simulink model "beaver_agent_env_ground_brake"  (R2022a)
settings: Solver=ode15s  StartTime=0.0  StopTime=30  FixedStep=1/120  MaxStep=0.005  RelTol=1e-6  AbsTol=1e-8
PreLoadFcn:
  | [aircraft, state] = astDehavillandBeaver();
  | thrustX = getCoefficient(aircraft,"CX","Propeller",Component="Propeller");
  | AileronCmd = 0.00202547955338193;
  | ElevatorCmd = -0.0109658218633661;
  | RudderCmd = -0.0374364069557001;
  | Throttle_Left = 0.16863024396043;
  | Throttle_Right = 0.16863024396043;
  | NoseWheelSteerCmdData = timeseries(0,0);
  | GearDownCmd = 1; RunwayMu = 0.65;
  | GroundMass = state.Mass;
  | GroundCrr = 0.015; GroundSideVGain = 0.35;
  | GroundYawGain = 0.15; GroundSteerGain = 0.8; NoseGearArm = 2.4;
  | 
  | Throttle_Left=0; Throttle_Right=0;
  | AileronCmd=0; ElevatorCmd=0; RudderCmd=0;
  | NoseWheelSteerCmdData=timeseries([0;0],[0;60]);
model workspace (MATLAB code in the model file + MAT data in the model file):
  GroundStatic.GearPositions = [2.4  0  1.5; -0.8  -1  1.5; -0.8  1  1.5]
  GroundStatic.RunwayZ = 0
  GroundStatic.StaticCompression = 0.06
  GroundStatic.InitialPosition = [0 0 -1.44]
  GroundStatic.InitialPositionOffset = [0 0 0]
  GroundStatic.InitialVelocity = [0 0 0]
  GroundStatic.InitialAttitude = [0 0 0]
  GroundStatic.InitialAngularRates = [0 0 0]
  GroundStatic.Mass = 2288.231
  GroundStatic.ReferenceGravity = 9.78032088963
  GroundStatic.LoadFractions = [0.25; 0.375; 0.375]
  GroundStatic.StaticWheelLoads = [5594.9083624; 8392.3625436; 8392.3625436]
  GroundStatic.NormalStiffness = [93248.4727066; 139872.70906; 139872.70906]
  GroundStatic.DampingRatio = 0.85
  GroundStatic.NormalDamping = [12416.2292263; 18624.3438394; 18624.3438394]
  GroundStatic.TireVelocityScale = 0.1
  GroundStatic.TireLateralCoefficient = 1
  GroundStatic.RollingCoefficient = 0.015
  GroundStatic.ParkingBrakeCoefficient = 0.5
  GroundStatic.ParkingBrakeCmd = 1
  GroundStatic.RunwayMu = 0.65
  GroundStatic.GearDown = 1
  GroundStatic.PowerOff = 1
  GroundStatic.AirSpeedFloor = 1
  GroundStatic.Description = 'Assumed three-point demonstration gear; replace with actual aircraft geometry/stiffness for performance use.'
  GroundStatic.LeftBrakeManual = 0
  GroundStatic.RightBrakeManual = 0
  GroundStatic.BrakeMode = 0
  GroundStatic.RunwayCenterlineYe = 0
  GroundStatic.RunwayCorrectionOnThreshold = 15.24
  GroundStatic.RunwayCorrectionOffThreshold = 3.048
  GroundStatic.RunwayCorrectionKp = 0.1
  GroundStatic.RunwayCorrectionKd = 0.5
  GroundStatic.DifferentialBrakeLimit = 1
  GroundStatic.BrakeCoefficient = 0.5
  GroundStatic.CorrectionRunwayAxis = 'Xe'
  GroundStatic.BrakeSystemMode = 1
  GroundStatic.AutoBrakePreArm = 0
  GroundStatic.AutoBrakeMinLevel = 0.15
  GroundStatic.NoseSteerLowSpeed = 2
  GroundStatic.NoseSteerHighSpeed = 20
  GroundStatic.NoseSteerAngleLowSpeed = 1.308996939
  GroundStatic.NoseSteerAngleHighSpeed = 0.10471975512
  inputs0.time = 0
  inputs0.signals(1).dimensions = 1
  inputs0.signals(1).values = -0.104711430294
  inputs0.signals(2).dimensions = 1
  inputs0.signals(2).values = -0.0698725229544
  inputs0.signals(3).dimensions = 1
  inputs0.signals(3).values = -0.000215042330254
  states.time = 0
  states.signals(1).values = 0
  states.signals(1).dimensions = 1
  states.signals(1).label = 'CSTATE'
  states.signals(1).blockName = 'untitled/6DOF EOM/6DOF (Euler Angles)/xe,ye,ze'
  states.signals(1).stateName = 'Xe'
  states.signals(1).inReferencedModel = 0
  states.signals(1).sampleTime = [0 0]
  states.signals(2).values = 0
  states.signals(2).dimensions = 1
  states.signals(2).label = 'CSTATE'
  states.signals(2).blockName = 'untitled/6DOF EOM/6DOF (Euler Angles)/xe,ye,ze'
  states.signals(2).stateName = 'Ye'
  states.signals(2).inReferencedModel = 0
  states.signals(2).sampleTime = [0 0]
  states.signals(3).values = -2202
  states.signals(3).dimensions = 1
  states.signals(3).label = 'CSTATE'
  states.signals(3).blockName = 'untitled/6DOF EOM/6DOF (Euler Angles)/xe,ye,ze'
  states.signals(3).stateName = 'Ze'
  states.signals(3).inReferencedModel = 0
  states.signals(3).sampleTime = [0 0]
  states.signals(4).values = 0.128665353089
  states.signals(4).dimensions = 1
  states.signals(4).label = 'CSTATE'
  states.signals(4).blockName = 'untitled/6DOF EOM/6DOF (Euler Angles)/Calculate DCM &
    | Euler Angles/phi
    | theta
    | psi'
  states.signals(4).stateName = 'phi'
  states.signals(4).inReferencedModel = 0
  states.signals(4).sampleTime = [0 0]
  states.signals(5).values = 0.259337659946
  states.signals(5).dimensions = 1
  states.signals(5).label = 'CSTATE'
  states.signals(5).blockName = 'untitled/6DOF EOM/6DOF (Euler Angles)/Calculate DCM &
    | Euler Angles/phi
    | theta
    | psi'
  states.signals(5).stateName = 'theta'
  states.signals(5).inReferencedModel = 0
  states.signals(5).sampleTime = [0 0]
  states.signals(6).values = -0.178947917154
  states.signals(6).dimensions = 1
  states.signals(6).label = 'CSTATE'
  states.signals(6).blockName = 'untitled/6DOF EOM/6DOF (Euler Angles)/Calculate DCM &
    | Euler Angles/phi
    | theta
    | psi'
  states.signals(6).stateName = 'psi'
  states.signals(6).inReferencedModel = 0
  states.signals(6).sampleTime = [0 0]
  states.signals(7).values = 36.9119692666
  states.signals(7).dimensions = 1
  states.signals(7).label = 'CSTATE'
  states.signals(7).blockName = 'untitled/6DOF EOM/6DOF (Euler Angles)/ub,vb,wb'
  states.signals(7).stateName = 'U'
  states.signals(7).inReferencedModel = 0
  states.signals(7).sampleTime = [0 0]
  states.signals(8).values = 8.10720863264
  states.signals(8).dimensions = 1
  states.signals(8).label = 'CSTATE'
  states.signals(8).blockName = 'untitled/6DOF EOM/6DOF (Euler Angles)/ub,vb,wb'
  states.signals(8).stateName = 'V'
  states.signals(8).inReferencedModel = 0
  states.signals(8).sampleTime = [0 0]
  states.signals(9).values = 8.82591882596
  states.signals(9).dimensions = 1
  states.signals(9).label = 'CSTATE'
  states.signals(9).blockName = 'untitled/6DOF EOM/6DOF (Euler Angles)/ub,vb,wb'
  states.signals(9).stateName = 'W'
  states.signals(9).inReferencedModel = 0
  states.signals(9).sampleTime = [0 0]
  states.signals(10).values = 0
  states.signals(10).dimensions = 1
  states.signals(10).label = 'CSTATE'
  states.signals(10).blockName = 'untitled/6DOF EOM/6DOF (Euler Angles)/p,q,r '
  states.signals(10).stateName = 'p'
  states.signals(10).inReferencedModel = 0
  states.signals(10).sampleTime = [0 0]
  states.signals(11).values = 0
  states.signals(11).dimensions = 1
  states.signals(11).label = 'CSTATE'
  states.signals(11).blockName = 'untitled/6DOF EOM/6DOF (Euler Angles)/p,q,r '
  states.signals(11).stateName = 'q'
  states.signals(11).inReferencedModel = 0
  states.signals(11).sampleTime = [0 0]
  states.signals(12).values = 0
  states.signals(12).dimensions = 1
  states.signals(12).label = 'CSTATE'
  states.signals(12).blockName = 'untitled/6DOF EOM/6DOF (Euler Angles)/p,q,r '
  states.signals(12).stateName = 'r'
  states.signals(12).inReferencedModel = 0
  states.signals(12).sampleTime = [0 0]
  states.signals(13).values = 0
  states.signals(13).dimensions = 1
  states.signals(13).label = 'CSTATE'
  states.signals(13).blockName = 'untitled/PID Controller/Integrator/Continuous/Integrator'
  states.signals(13).stateName = ''
  states.signals(13).inReferencedModel = 0
  states.signals(13).sampleTime = [0 0]
  states.signals(14).values = 0
  states.signals(14).dimensions = 1
  states.signals(14).label = 'CSTATE'
  states.signals(14).blockName = 'untitled/PID Controller/Filter/Cont. Filter/Filter'
  states.signals(14).stateName = ''
  states.signals(14).inReferencedModel = 0
  states.signals(14).sampleTime = [0 0]
  states.signals(15).values = 0
  states.signals(15).dimensions = 1
  states.signals(15).label = 'CSTATE'
  states.signals(15).blockName = 'untitled/PID Controller1/Integrator/Continuous/Integrator'
  states.signals(15).stateName = ''
  states.signals(15).inReferencedModel = 0
  states.signals(15).sampleTime = [0 0]
  states.signals(16).values = 0
  states.signals(16).dimensions = 1
  states.signals(16).label = 'CSTATE'
  states.signals(16).blockName = 'untitled/PID Controller1/Filter/Cont. Filter/Filter'
  states.signals(16).stateName = ''
  states.signals(16).inReferencedModel = 0
  states.signals(16).sampleTime = [0 0]
  states.signals(17).values = [0 0]
  states.signals(17).dimensions = 2
  states.signals(17).label = 'CSTATE'
  states.signals(17).blockName = 'untitled/Environment Model/Dryden Wind Turbulence Model 
    | (Continuous (+q +r))/Filters on velocities/Hwgw(s)/wg_p1'
  states.signals(17).stateName = ''
  states.signals(17).inReferencedModel = 0
  states.signals(17).sampleTime = [0 0]
  states.signals(18).values = [0 0]
  states.signals(18).dimensions = 2
  states.signals(18).label = 'CSTATE'
  states.signals(18).blockName = 'untitled/Environment Model/Dryden Wind Turbulence Model 
    | (Continuous (+q +r))/Filters on velocities/Hwgw(s)/wg_p2'
  states.signals(18).stateName = ''
  states.signals(18).inReferencedModel = 0
  states.signals(18).sampleTime = [0 0]
  states.signals(19).values = [0 0]
  states.signals(19).dimensions = 2
  states.signals(19).label = 'CSTATE'
  states.signals(19).blockName = 'untitled/Environment Model/Dryden Wind Turbulence Model 
    | (Continuous (+q +r))/Filters on velocities/Hvgw(s)/vg_p1'
  states.signals(19).stateName = ''
  states.signals(19).inReferencedModel = 0
  states.signals(19).sampleTime = [0 0]
  states.signals(20).values = [0 0]
  states.signals(20).dimensions = 2
  states.signals(20).label = 'CSTATE'
  states.signals(20).blockName = 'untitled/Environment Model/Dryden Wind Turbulence Model 
    | (Continuous (+q +r))/Filters on velocities/Hvgw(s)/vgw_p2'
  states.signals(20).stateName = ''
  states.signals(20).inReferencedModel = 0
  states.signals(20).sampleTime = [0 0]
  states.signals(21).values = [0 0]
  states.signals(21).dimensions = 2
  states.signals(21).label = 'CSTATE'
  states.signals(21).blockName = 'untitled/Environment Model/Dryden Wind Turbulence Model 
    | (Continuous (+q +r))/Filters on velocities/Hugw(s)/ug_p'
  states.signals(21).stateName = ''
  states.signals(21).inReferencedModel = 0
  states.signals(21).sampleTime = [0 0]
  states.signals(22).values = [0 0]
  states.signals(22).dimensions = 2
  states.signals(22).label = 'CSTATE'
  states.signals(22).blockName = 'untitled/Environment Model/Dryden Wind Turbulence Model 
    | (Continuous (+q +r))/Filters on angular rates/Hrgw/rgw_p'
  states.signals(22).stateName = ''
  states.signals(22).inReferencedModel = 0
  states.signals(22).sampleTime = [0 0]
  states.signals(23).values = [0 0]
  states.signals(23).dimensions = 2
  states.signals(23).label = 'CSTATE'
  states.signals(23).blockName = 'untitled/Environment Model/Dryden Wind Turbulence Model 
    | (Continuous (+q +r))/Filters on angular rates/Hqgw/qgw_p'
  states.signals(23).stateName = ''
  states.signals(23).inReferencedModel = 0
  states.signals(23).sampleTime = [0 0]
  states.signals(24).values = [0 0]
  states.signals(24).dimensions = 2
  states.signals(24).label = 'CSTATE'
  states.signals(24).blockName = 'untitled/Environment Model/Dryden Wind Turbulence Model 
    | (Continuous (+q +r))/Filters on angular rates/Hpgw/pgw_p'
  states.signals(24).stateName = ''
  states.signals(24).inReferencedModel = 0
  states.signals(24).sampleTime = [0 0]
  states0.time = 0
  states0.signals(1).values = [0 0 -2202]
  states0.signals(1).dimensions = 3
  states0.signals(1).label = 'CSTATE'
  states0.signals(1).blockName = 'asb6DOFAirframeTemplate/6DOF EOM/6DOF (Euler Angles)/xe,ye,ze'
  states0.signals(1).stateName = ''
  states0.signals(1).inReferencedModel = 0
  states0.signals(1).sampleTime = [0 0]
  states0.signals(2).values = [0.128665353089 0.259337659946 -0.178947917154]
  states0.signals(2).dimensions = 3
  states0.signals(2).label = 'CSTATE'
  states0.signals(2).blockName = 'asb6DOFAirframeTemplate/6DOF EOM/6DOF (Euler Angles)/Calculate DCM &
    | Euler Angles/phi
    | theta
    | psi'
  states0.signals(2).stateName = ''
  states0.signals(2).inReferencedModel = 0
  states0.signals(2).sampleTime = [0 0]
  states0.signals(3).values = [36.9119692666 8.10720863264 8.82591882596]
  states0.signals(3).dimensions = 3
  states0.signals(3).label = 'CSTATE'
  states0.signals(3).blockName = 'asb6DOFAirframeTemplate/6DOF EOM/6DOF (Euler Angles)/ub,vb,wb'
  states0.signals(3).stateName = ''
  states0.signals(3).inReferencedModel = 0
  states0.signals(3).sampleTime = [0 0]
  states0.signals(4).values = [0 0 0]
  states0.signals(4).dimensions = 3
  states0.signals(4).label = 'CSTATE'
  states0.signals(4).blockName = 'asb6DOFAirframeTemplate/6DOF EOM/6DOF (Euler Angles)/p,q,r '
  states0.signals(4).stateName = ''
  states0.signals(4).inReferencedModel = 0
  states0.signals(4).sampleTime = [0 0]
  states0.signals(5).values = [0 0]
  states0.signals(5).dimensions = 2
  states0.signals(5).label = 'CSTATE'
  states0.signals(5).blockName = 'asb6DOFAirframeTemplate/Environment Model/Dryden Wind Turbulence Model 
    | (Continuous (+q +r))/Filters on velocities/Hwgw(s)/wg_p1'
  states0.signals(5).stateName = ''
  states0.signals(5).inReferencedModel = 0
  states0.signals(5).sampleTime = [0 0]
  states0.signals(6).values = [0 0]
  states0.signals(6).dimensions = 2
  states0.signals(6).label = 'CSTATE'
  states0.signals(6).blockName = 'asb6DOFAirframeTemplate/Environment Model/Dryden Wind Turbulence Model 
    | (Continuous (+q +r))/Filters on velocities/Hwgw(s)/wg_p2'
  states0.signals(6).stateName = ''
  states0.signals(6).inReferencedModel = 0
  states0.signals(6).sampleTime = [0 0]
  states0.signals(7).values = [0 0]
  states0.signals(7).dimensions = 2
  states0.signals(7).label = 'CSTATE'
  states0.signals(7).blockName = 'asb6DOFAirframeTemplate/Environment Model/Dryden Wind Turbulence Model 
    | (Continuous (+q +r))/Filters on velocities/Hvgw(s)/vg_p1'
  states0.signals(7).stateName = ''
  states0.signals(7).inReferencedModel = 0
  states0.signals(7).sampleTime = [0 0]
  states0.signals(8).values = [0 0]
  states0.signals(8).dimensions = 2
  states0.signals(8).label = 'CSTATE'
  states0.signals(8).blockName = 'asb6DOFAirframeTemplate/Environment Model/Dryden Wind Turbulence Model 
    | (Continuous (+q +r))/Filters on velocities/Hvgw(s)/vgw_p2'
  states0.signals(8).stateName = ''
  states0.signals(8).inReferencedModel = 0
  states0.signals(8).sampleTime = [0 0]
  states0.signals(9).values = [0 0]
  states0.signals(9).dimensions = 2
  states0.signals(9).label = 'CSTATE'
  states0.signals(9).blockName = 'asb6DOFAirframeTemplate/Environment Model/Dryden Wind Turbulence Model 
    | (Continuous (+q +r))/Filters on velocities/Hugw(s)/ug_p'
  states0.signals(9).stateName = ''
  states0.signals(9).inReferencedModel = 0
  states0.signals(9).sampleTime = [0 0]
  states0.signals(10).values = [0 0]
  states0.signals(10).dimensions = 2
  states0.signals(10).label = 'CSTATE'
  states0.signals(10).blockName = 'asb6DOFAirframeTemplate/Environment Model/Dryden Wind Turbulence Model 
    | (Continuous (+q +r))/Filters on angular rates/Hrgw/rgw_p'
  states0.signals(10).stateName = ''
  states0.signals(10).inReferencedModel = 0
  states0.signals(10).sampleTime = [0 0]
  states0.signals(11).values = [0 0]
  states0.signals(11).dimensions = 2
  states0.signals(11).label = 'CSTATE'
  states0.signals(11).blockName = 'asb6DOFAirframeTemplate/Environment Model/Dryden Wind Turbulence Model 
    | (Continuous (+q +r))/Filters on angular rates/Hqgw/qgw_p'
  states0.signals(11).stateName = ''
  states0.signals(11).inReferencedModel = 0
  states0.signals(11).sampleTime = [0 0]
  states0.signals(12).values = [0 0]
  states0.signals(12).dimensions = 2
  states0.signals(12).label = 'CSTATE'
  states0.signals(12).blockName = 'asb6DOFAirframeTemplate/Environment Model/Dryden Wind Turbulence Model 
    | (Continuous (+q +r))/Filters on angular rates/Hpgw/pgw_p'
  states0.signals(12).stateName = ''
  states0.signals(12).inReferencedModel = 0
  states0.signals(12).sampleTime = [0 0]
  other statements: initialize6DOFSkyHogg;
values from neighbouring files (symbols this model uses):
  r = vec(out.r)    [ground_realtime_worker.m]    (also in probe_brake_correction.m; verify_ground_brake_model.m = runCase('turn_right_10',g,10,8))
  state = squeeze(controls.Data)    [finalize_ground_capability_checks.m]    (also in run_ground_capability_checks.m)
undefined symbols (not defined in the file or in its folder): aircraft, Earth, F, Light, MIL, WGS84
libraries: simulink x5, shared6dof x1, aerolibadyn x1, aerolibasang x1, aerolibatmos2 x1, aerolibwind2 x1, aerolibtransform2 x1, sharedtransform x1
(part 1 of 3)
settings Model: Creator=Petrichor  LastModifiedBy=velpro
settings SolverCC: AlgebraicLoopSolver=TrustRegion  AutoInsertRateTranBlk=on  InsertRTBMode=Never (minimum delay)  MinimalZcImpactIntegration=on  MaxZcPerStep=1
settings DataIOCC: ExternalInput=inputs0  InitialState=states  SaveFinalState=on  SaveFormat=Array  SaveState=on  LoggingToFile=on
settings OptimizationCC: EnhancedBackFolding=on  StrengthReduction=on  InitFltsAndDblsToZero=on  DifferentSizesBufferReuse=on
settings DebuggingCC: WriteAfterWriteMsg=DisableAll  AlgebraicLoopMsg=none  FcnCallInpInsideContextMsg=warning  UniqueDataStoreMsg=error  RootOutportRequireBusObject=none  StateNameClashWarn=warning  StrictBusMsg=ErrorOnBusTreatedAsVector  SFUnexpectedBacktrackingDiag=warning  SFNoUnconditionalDefaultTransitionDiag=warning  SFExecutionAtInitializationDiag=none  SFMachineParentedDataDiag=warning  ArithmeticOperatorsInVariantConditions=warning
settings ModelReferenceCC: PropagateSignalLabelsOutOfModel=off
settings SFSimCC: SimUseLocalCustomCode=off
settings RTWCC: RTWUseLocalCustomCode=off  DLArmComputeVersion=19.05
settings CodeAppCC: StateflowObjectComments=on

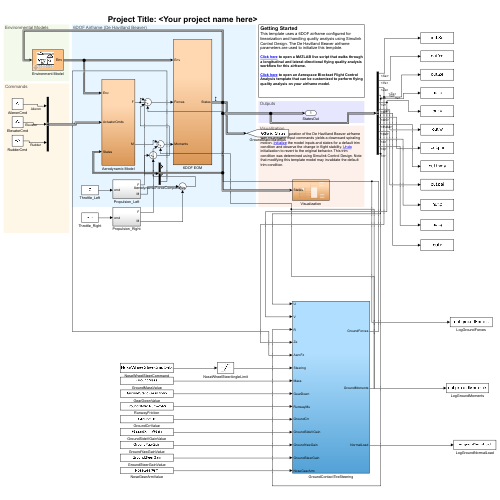
[thumbnail: Simulink's stored preview of the top-level diagram]
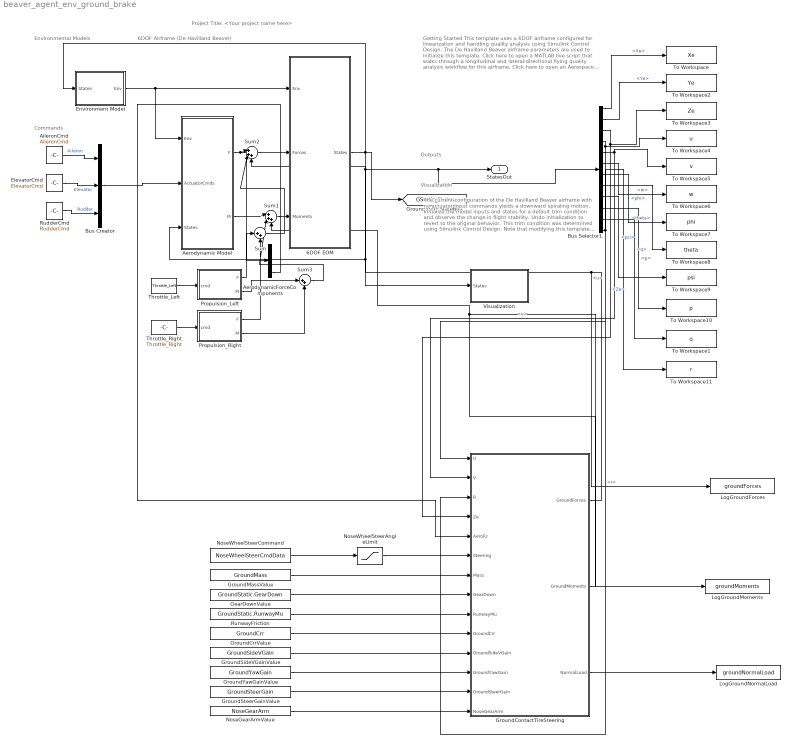
== system beaver_agent_env_ground_brake ==
  note: Project Title: <Your project name here>
  note: 6DOF Airframe (De Havilland Beaver)
  note: Environmental Models
  note: Commands
  note: The current configuration of the De Havilland Beaver airframe with no actuator input commands yields a downward spiraling motion. Initialize the model inputs and states for a default trim condition and observe the change in flight stability. Undo initialization to revert to the original behavior. This trim condition was determined using Simulink Control Design. Note that modifying this template model may invalidate the default trim condition.
  note: Visualization
  note: Outputs
  note: Getting Started
      | This template uses a 6DOF airframe configured for linearization and handling quality analysis using Simulink Control Design. The De Havilland Beaver airframe parameters are used to initialize this template.
      |
      | Click here to open a MATLAB live script that walks through a longitudinal and lateral-directional flying quality analysis workflow for this airframe.
      |
      | Click here to open an Aerospace Blockset Flight Control Analysis template that can be customized to perform flying quality analysis on your airframe model.
  6DOF EOM : Subsystem  VariantControl=eom3DOF
  Aerodynamic Model : Subsystem  VariantControl=aeroCONST
  AerodynamicForceComponents : Demux  Outputs=3
  AileronCmd : Constant  Value=AileronCmd
  Bus Creator : BusCreator  Inputs=3
  Bus Selector1 : BusSelector  OutputSignals=Xe,Ye,Ze,u,v,w,phi,theta,psi,p,q,r
  ElevatorCmd : Constant  Value=ElevatorCmd
  Environment Model : Subsystem  mask(Environment Model){spec=MIL-F-8785C, model=Continuous Dryden (+q -r), W20=5, Wdeg=0, TurbProb=10^-2 - Light, L_high=533.4, Wingspan=4, ts=0.1, Seed=[23341 23342 23343 23344], T_on=off, refAlt=state.GroundHeight}
      mask prompts: spec "aeroblks:aeroblkwind:blockWindTurbulenceModelParamSpecification"; model "aeroblks:aeroblkwind:blockWindTurbulenceModelParamModeltype"; W20 "Wind speed at 6 m defines the low-altitude intensity (m/s):"; Wdeg "Wind direction at 6 m (degrees clockwise from north):"; TurbProb "aeroblks:aeroblkwind:blockWindTurbulenceModelParamProbabilityofexceedanceofhighaltitudeintensity"; L_high "Scale length at medium/high altitudes (m):"; Wingspan "Wingspan (m):"; ts "Band limited noise sample time (sec):"; Seed "aeroblks:aeroblkwind:blockWindTurbulenceModelParamNoiseseedsugvgwgpg"; T_on "aeroblks:aeroblkwind:blockWindTurbulenceModelParamTurbulenceon"; refAlt "Reference height from Earth's surface to Flat Earth frame [m]:"
      mask help: This block contains an athmospheric model, a wind turbulence model, and a gravity model.
      mask Help: helpview(fullfile(docroot,'toolbox','aeroblks','aeroblks.map'), 'environment1');
      mask TypeOptions spec:
      | Dryden Wind Turbulence Model
      | (Continuous (+q +r))/spec
      mask TypeOptions model:
      | Dryden Wind Turbulence Model
      | (Continuous (+q +r))/model
      mask TypeOptions W20:
      | Dryden Wind Turbulence Model
      | (Continuous (+q +r))/W20
      mask TypeOptions Wdeg:
      | Dryden Wind Turbulence Model
      | (Continuous (+q +r))/Wdeg
      mask TypeOptions TurbProb:
      | Dryden Wind Turbulence Model
      | (Continuous (+q +r))/TurbProb
      mask TypeOptions L_high:
      | Dryden Wind Turbulence Model
      | (Continuous (+q +r))/L_high
      mask TypeOptions Wingspan:
      | Dryden Wind Turbulence Model
      | (Continuous (+q +r))/Wingspan
      mask TypeOptions ts:
      | Dryden Wind Turbulence Model
      | (Continuous (+q +r))/ts
      mask TypeOptions Seed:
      | Dryden Wind Turbulence Model
      | (Continuous (+q +r))/Seed
      mask TypeOptions T_on:
      | Dryden Wind Turbulence Model
      | (Continuous (+q +r))/T_on
      mask DialogControl Container4 Prompt: Atmospheric Model
      mask DialogControl Container17 Prompt: 1976 COESA-extended U.S. Standard Atmospheric Model
      mask DialogControl Control6 Prompt: There are no modifiable parameters for COESA.
      mask DialogControl Container6 Prompt: Wind Model
      mask DialogControl Container16 Prompt: Dryden Wind Turbulence Model
      mask DialogControl spec Prompt: Specification:
      mask DialogControl model Prompt: Model type:
      mask DialogControl TurbProb Prompt: Probability of exceedance of high-altitude intensity:
      mask DialogControl Seed Prompt: Noise seeds [ug vg wg pg]:
      mask DialogControl T_on Prompt: Turbulence on
      mask DialogControl Container8 Prompt: Gravity Model
      mask DialogControl Container18 Prompt: World Geodetic System (WGS 84) Gravity Taylor Series Model
      mask Display:
      | image('aeroenvironment.bmp',[.15,.15,.55,.75])
      | port_label('output',1,'Env')
  GearDownValue : Constant  Value=GroundStatic.GearDown
  GroundContactTireSteering : Subsystem
  GroundCrrValue : Constant  Value=GroundCrr
  GroundMassValue : Constant  Value=GroundMass
  GroundSideVGainValue : Constant  Value=GroundSideVGain
  GroundSteerGainValue : Constant  Value=GroundSteerGain
  GroundYawGainValue : Constant  Value=GroundYawGain
  LogGroundForces : ToWorkspace  VariableName=groundForces  SaveFormat=Timeseries  SampleTime=-1
  LogGroundMoments : ToWorkspace  VariableName=groundMoments  SaveFormat=Timeseries  SampleTime=-1
  LogGroundNormalLoad : ToWorkspace  VariableName=groundNormalLoad  SaveFormat=Timeseries  SampleTime=-1
  NoseGearArmValue : Constant  Value=NoseGearArm
  NoseWheelSteerAngleLimit : Saturate  UpperLimit=1.308996939  LowerLimit=-1.308996939
  NoseWheelSteerCommand : FromWorkspace  VariableName=NoseWheelSteerCmdData  Interpolate=off  OutputAfterFinalValue=Holding final value
  Propulsion_Left : Subsystem
      settings: RTWSystemCode=Inline
  Propulsion_Right : Subsystem
      settings: RTWSystemCode=Inline
  RudderCmd : Constant  Value=RudderCmd
  RunwayFriction : Constant  Value=GroundStatic.RunwayMu
  Sum : Sum  Inputs=|++
  Sum1 : Sum  Inputs=|+++  InputSameDT=on  SaturateOnIntegerOverflow=on  OutDataTypeStr=Inherit: Same as first input
  Sum2 : Sum  Inputs=|+++  InputSameDT=on  SaturateOnIntegerOverflow=on  OutDataTypeStr=Inherit: Same as first input
  Sum3 : Sum  Inputs=|++
  Throttle_Left : Constant  Value=Throttle_Left
  Throttle_Right : Constant  Value=Throttle_Right
  To Workspace : ToWorkspace  VariableName=Xe  SaveFormat=Timeseries  SampleTime=-1
  To Workspace1 : ToWorkspace  VariableName=q  SaveFormat=Timeseries  SampleTime=-1
  To Workspace10 : ToWorkspace  VariableName=p  SaveFormat=Timeseries  SampleTime=-1
  To Workspace11 : ToWorkspace  VariableName=r  SaveFormat=Timeseries  SampleTime=-1
  To Workspace2 : ToWorkspace  VariableName=Ye  SaveFormat=Timeseries  SampleTime=-1
  To Workspace3 : ToWorkspace  VariableName=Ze  SaveFormat=Timeseries  SampleTime=-1
  To Workspace4 : ToWorkspace  VariableName=u  SaveFormat=Timeseries  SampleTime=-1
  To Workspace5 : ToWorkspace  VariableName=v  SaveFormat=Timeseries  SampleTime=-1
  To Workspace6 : ToWorkspace  VariableName=w  SaveFormat=Timeseries  SampleTime=-1
  To Workspace7 : ToWorkspace  VariableName=phi  SaveFormat=Timeseries  SampleTime=-1
  To Workspace8 : ToWorkspace  VariableName=theta  SaveFormat=Timeseries  SampleTime=-1
  To Workspace9 : ToWorkspace  VariableName=psi  SaveFormat=Timeseries  SampleTime=-1
  Visualization : Subsystem
  StatesOut : Outport  OutDataTypeStr=double  VectorParamsAs1DForOutWhenUnconnected=off
  tag scope: GStatic_States=global
  wires:
  AileronCmd/1 -> Bus Creator/1  "Aileron"
  RudderCmd/1 -> Bus Creator/3  "Rudder"
  Sum2/1 -> 6DOF EOM/2(Forces)
  Sum1/1 -> 6DOF EOM/3(Moments)
  Aerodynamic Model/1(F) -> Sum2/1, AerodynamicForceComponents/1
  Aerodynamic Model/2(M) -> Sum1/1
  Environment Model/1(Env) -> 6DOF EOM/1(Env), Aerodynamic Model/1(Env)
  Bus Creator/1 -> Aerodynamic Model/2(ActuatorCmds)
  Propulsion_Left/1(F) -> Sum/1
  Propulsion_Right/1(F) -> Sum/2
  Sum/1 -> Sum2/2
  Propulsion_Left/2(M) -> Sum3/1
  Propulsion_Right/2(M) -> Sum3/2
  Sum3/1 -> Sum1/2
  ElevatorCmd/1 -> Bus Creator/2  "Elevator"
  Throttle_Left/1 -> Propulsion_Left/1(cmd)
  Throttle_Right/1 -> Propulsion_Right/1(cmd)
  Bus Selector1/4 -> To Workspace4/1, GroundContactTireSteering/1(U)  "<u>"
  Bus Selector1/6 -> To Workspace6/1  "<w>"
  Bus Selector1/10 -> To Workspace10/1  "<p>"
  Bus Selector1/11 -> To Workspace1/1  "<q>"
  Bus Selector1/7 -> To Workspace7/1  "<phi>"
  Bus Selector1/1 -> To Workspace/1  "<Xe>"
  Bus Selector1/9 -> To Workspace9/1  "<psi>"
  Bus Selector1/2 -> To Workspace2/1  "<Ye>"
  6DOF EOM/1(States) -> [GStatic_States], Environment Model/1(States), Bus Selector1/1, StatesOut/1, Aerodynamic Model/3(States), Visualization/1(States)
  Bus Selector1/8 -> To Workspace8/1  "<theta>"
  Bus Selector1/12 -> To Workspace11/1, GroundContactTireSteering/3(R)  "<r>"
  Bus Selector1/5 -> To Workspace5/1, GroundContactTireSteering/2(V)  "<v>"
  Bus Selector1/3 -> To Workspace3/1, GroundContactTireSteering/4(Ze)  "<Ze>"
  NoseWheelSteerCommand/1 -> NoseWheelSteerAngleLimit/1
  AerodynamicForceComponents/3 -> GroundContactTireSteering/5(AeroFz)
  NoseWheelSteerAngleLimit/1 -> GroundContactTireSteering/6(Steering)
  GroundMassValue/1 -> GroundContactTireSteering/7(Mass)
  GearDownValue/1 -> GroundContactTireSteering/8(GearDown)
  RunwayFriction/1 -> GroundContactTireSteering/9(RunwayMu)
  GroundCrrValue/1 -> GroundContactTireSteering/10(GroundCrr)
  GroundSideVGainValue/1 -> GroundContactTireSteering/11(GroundSideVGain)
  GroundYawGainValue/1 -> GroundContactTireSteering/12(GroundYawGain)
  GroundSteerGainValue/1 -> GroundContactTireSteering/13(GroundSteerGain)
  NoseGearArmValue/1 -> GroundContactTireSteering/14(NoseGearArm)
  GroundContactTireSteering/1(GroundForces) -> Sum2/3, LogGroundForces/1
  GroundContactTireSteering/2(GroundMoments) -> Sum1/3, LogGroundMoments/1
  GroundContactTireSteering/3(NormalLoad) -> LogGroundNormalLoad/1

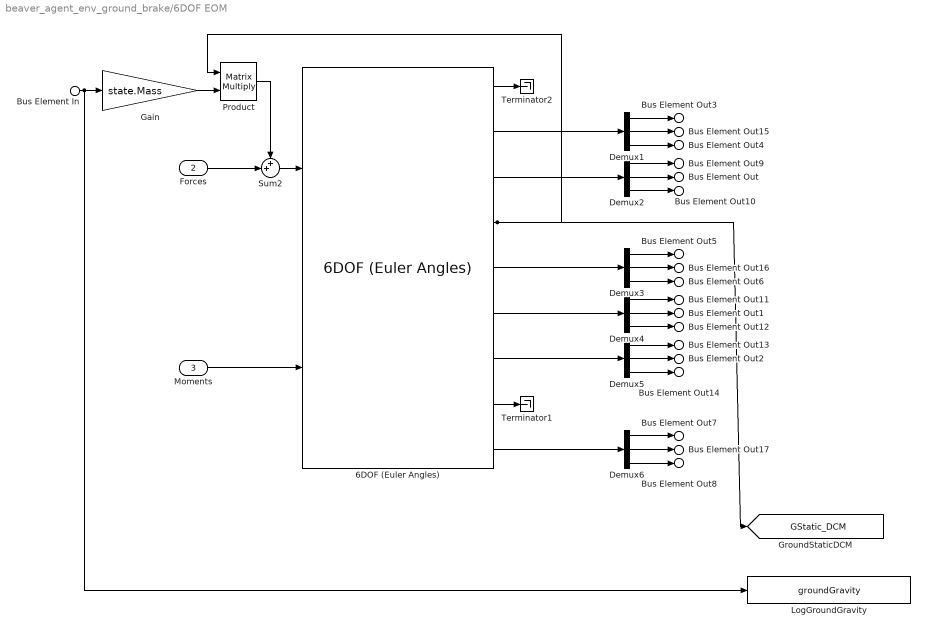
== system beaver_agent_env_ground_brake/6DOF EOM ==
  Bus Element In : Inport  PortName=Env  Element=g
  Forces : Inport  Port=2
  Moments : Inport  Port=3
  6DOF (Euler Angles) : shared6dof/6DOF (Euler Angles)  units=Metric (MKS)  mtype=Fixed  rep=Euler Angles  xme_0=GroundStatic.InitialPosition+GroundStatic.InitialPositionOffset  Vm_0=GroundStatic.InitialVelocity  eul_0=GroundStatic.InitialAttitude  pm_0=GroundStatic.InitialAngularRates  mass_0=state.Mass  mass_e=0.5  mass_f=2.0  inertia=state.Inertia.Variables  inertia_e=eye(3)  inertia_f=2*eye(3)  k_quat=1.0  vre_flag=on  abi_flag=on  aMode=0  xme_statename={'Xe', 'Ye', 'Ze'}  Vm_statename={'U', 'V', 'W'}  eul_statename={'phi', 'theta', 'psi'}  quat_statename={'qr', 'qi', 'qj','qk'}  pm_statename={'p', 'q', 'r'}  mass_statename=''
      settings: SourceProductBaseCode=AE,PW,DR,MT,VE
  Demux{1..6} (6 alike) : Demux  Outputs=3
  Gain : Gain  Gain=state.Mass
  LogGroundGravity : ToWorkspace  VariableName=groundGravity  SaveFormat=Timeseries  SampleTime=-1
  Product : Product  Multiplication=Matrix(*)
  Sum2 : Sum  Inputs=++|  InputSameDT=on  SaturateOnIntegerOverflow=on  OutDataTypeStr=Inherit: Same as first input
  Terminator1 : Terminator
  Terminator2 : Terminator
  Bus Element Out3 : Outport  VectorParamsAs1DForOutWhenUnconnected=off  PortName=States  Element=Xe
  Bus Element Out4 : Outport  VectorParamsAs1DForOutWhenUnconnected=off  PortName=States  Element=Ze
  Bus Element Out : Outport  VectorParamsAs1DForOutWhenUnconnected=off  PortName=States  Element=theta
  Bus Element Out5 : Outport  VectorParamsAs1DForOutWhenUnconnected=off  PortName=States  Element=u
  Bus Element Out6 : Outport  VectorParamsAs1DForOutWhenUnconnected=off  PortName=States  Element=w
  Bus Element Out1 : Outport  VectorParamsAs1DForOutWhenUnconnected=off  PortName=States  Element=q
  Bus Element Out2 : Outport  VectorParamsAs1DForOutWhenUnconnected=off  PortName=States  Element=q_dot
  Bus Element Out7 : Outport  VectorParamsAs1DForOutWhenUnconnected=off  PortName=States  Element=Axe
  Bus Element Out8 : Outport  VectorParamsAs1DForOutWhenUnconnected=off  PortName=States  Element=Aze
  Bus Element Out15 : Outport  VectorParamsAs1DForOutWhenUnconnected=off  PortName=States  Element=Ye
  Bus Element Out9 : Outport  VectorParamsAs1DForOutWhenUnconnected=off  PortName=States  Element=phi
  Bus Element Out10 : Outport  VectorParamsAs1DForOutWhenUnconnected=off  PortName=States  Element=psi
  Bus Element Out16 : Outport  VectorParamsAs1DForOutWhenUnconnected=off  PortName=States  Element=v
  Bus Element Out11 : Outport  VectorParamsAs1DForOutWhenUnconnected=off  PortName=States  Element=p
  Bus Element Out12 : Outport  VectorParamsAs1DForOutWhenUnconnected=off  PortName=States  Element=r
  Bus Element Out13 : Outport  VectorParamsAs1DForOutWhenUnconnected=off  PortName=States  Element=p_dot
  Bus Element Out14 : Outport  VectorParamsAs1DForOutWhenUnconnected=off  PortName=States  Element=r_dot
  Bus Element Out17 : Outport  VectorParamsAs1DForOutWhenUnconnected=off  PortName=States  Element=Aye
  tag scope: GStatic_DCM=global
  wires:
  6DOF (Euler Angles)/2 -> Demux1/1
  6DOF (Euler Angles)/4 -> Product/1, [GStatic_DCM]
  6DOF (Euler Angles)/1 -> Terminator2/1
  Bus Element In/1 -> Gain/1, LogGroundGravity/1
  Demux6/2 -> Bus Element Out17/1
  Demux6/3 -> Bus Element Out8/1
  Demux6/1 -> Bus Element Out7/1
  6DOF (Euler Angles)/9 -> Demux6/1
  6DOF (Euler Angles)/7 -> Demux5/1
  Demux5/3 -> Bus Element Out14/1
  Demux5/2 -> Bus Element Out2/1
  Demux5/1 -> Bus Element Out13/1
  6DOF (Euler Angles)/6 -> Demux4/1
  Demux4/3 -> Bus Element Out12/1
  Demux4/2 -> Bus Element Out1/1
  Demux4/1 -> Bus Element Out11/1
  Demux3/3 -> Bus Element Out6/1
  Demux3/2 -> Bus Element Out16/1
  Demux3/1 -> Bus Element Out5/1
  6DOF (Euler Angles)/5 -> Demux3/1
  Demux2/3 -> Bus Element Out10/1
  Demux2/2 -> Bus Element Out/1
  Demux2/1 -> Bus Element Out9/1
  Demux1/1 -> Bus Element Out3/1
  Demux1/3 -> Bus Element Out4/1
  Demux1/2 -> Bus Element Out15/1
  Gain/1 -> Product/2
  6DOF (Euler Angles)/3 -> Demux2/1
  Moments/1 -> 6DOF (Euler Angles)/2
  Forces/1 -> Sum2/2
  Sum2/1 -> 6DOF (Euler Angles)/1
  Product/1 -> Sum2/1
  6DOF (Euler Angles)/8 -> Terminator1/1

== system beaver_agent_env_ground_brake/Aerodynamic Model ==
  note: De Havilland Beaver Aerodynamic Model
      | Based on original work created by
      | Marc Rauw for Delft University of Technology
      | http://www.dutchroll.com
  Bus Element In13 : Inport  PortName=Env  Element=AirDensity
  Bus Element In14 : Inport  PortName=Env  Element=WindVelocity
  Bus Element In15 : Inport  PortName=Env  Element=WindAngularRates
  ActuatorCmds : Inport  Port=2
  Bus Element In1 : Inport  Port=3  PortName=States  Element=u
  Bus Element In2 : Inport  Port=3  PortName=States  Element=w
  Bus Element In3 : Inport  Port=3  PortName=States  Element=q
  Bus Element In6 : Inport  Port=3  PortName=States  Element=v
  Bus Element In4 : Inport  Port=3  PortName=States  Element=p
  Bus Element In5 : Inport  Port=3  PortName=States  Element=r
  Actuator Aerodynamic Coefficients : Subsystem
  Aerodynamic Coefficients : Subsystem
  Aerodynamic Forces and Moments : aerolibadyn/Aerodynamic Forces and Moments   inputAxes=Body  outputForceAxes=Body  outputMomentAxes=Body  S=aircraft.ReferenceArea  b=aircraft.ReferenceSpan  cbar=aircraft.ReferenceLength
  Constant1 : Constant  Value=state.CenterOfGravity
  Constant2 : Constant  Value=state.CenterOfPressure
  Dynamic Pressure : aerolibasang/Dynamic Pressure
  Mux1 : Mux  Inputs=3
  Mux2 : Mux  Inputs=3
  Subsystem : Subsystem
  Sum1 : Sum  Inputs=-+|  InputSameDT=on  SaturateOnIntegerOverflow=on  OutDataTypeStr=Inherit: Same as first input
  Sum2 : Sum  Inputs=++|
  Sum3 : Sum  Inputs=|++  InputSameDT=on  SaturateOnIntegerOverflow=on  OutDataTypeStr=Inherit: Same as first input
  ToBus : Subsystem
  F : Outport  Unit=N  VectorParamsAs1DForOutWhenUnconnected=off
  M : Outport  Port=2  Unit=N*m  VectorParamsAs1DForOutWhenUnconnected=off
  wires:
  ActuatorCmds/1 -> Actuator Aerodynamic Coefficients/1(ActuatorCmds)
  Bus Element In14/1 -> Sum1/1
  Mux2/1 -> Sum1/2
  Mux1/1 -> Sum3/2
  Bus Element In15/1 -> Sum3/1
  Bus Element In5/1 -> Mux1/3
  Bus Element In3/1 -> Mux1/2
  Bus Element In4/1 -> Mux1/1
  Actuator Aerodynamic Coefficients/1(Coeff) -> Sum2/1
  Aerodynamic Coefficients/1(Coeff) -> Sum2/2
  ToBus/1(O) -> Aerodynamic Coefficients/8(pqr)
  Sum1/1 -> Dynamic Pressure/1, Subsystem/1(Vb)
  Dynamic Pressure/1 -> Aerodynamic Forces and Moments/2  "qbar"
  Sum3/1 -> ToBus/1(I)
  Bus Element In13/1 -> Dynamic Pressure/2
  Subsystem/7(V) -> Aerodynamic Coefficients/7(V)
  Subsystem/4(Beta) -> Aerodynamic Coefficients/4(Beta)
  Aerodynamic Forces and Moments/2 -> M/1
  Aerodynamic Forces and Moments/1 -> F/1
  Constant2/1 -> Aerodynamic Forces and Moments/4
  Constant1/1 -> Aerodynamic Forces and Moments/3
  Sum2/1 -> Aerodynamic Forces and Moments/1
  Bus Element In1/1 -> Mux2/1
  Bus Element In6/1 -> Mux2/2
  Bus Element In2/1 -> Mux2/3
  Subsystem/1(Alpha) -> Aerodynamic Coefficients/1(Alpha), Actuator Aerodynamic Coefficients/2(Alpha)
  Subsystem/5(Beta2) -> Aerodynamic Coefficients/5(Beta2), Actuator Aerodynamic Coefficients/3(Beta2)
  Subsystem/2(Alpha2) -> Aerodynamic Coefficients/2(Alpha2)
  Subsystem/3(Alpha3) -> Aerodynamic Coefficients/3(Alpha3)
  Subsystem/6(Beta3) -> Aerodynamic Coefficients/6(Beta3)

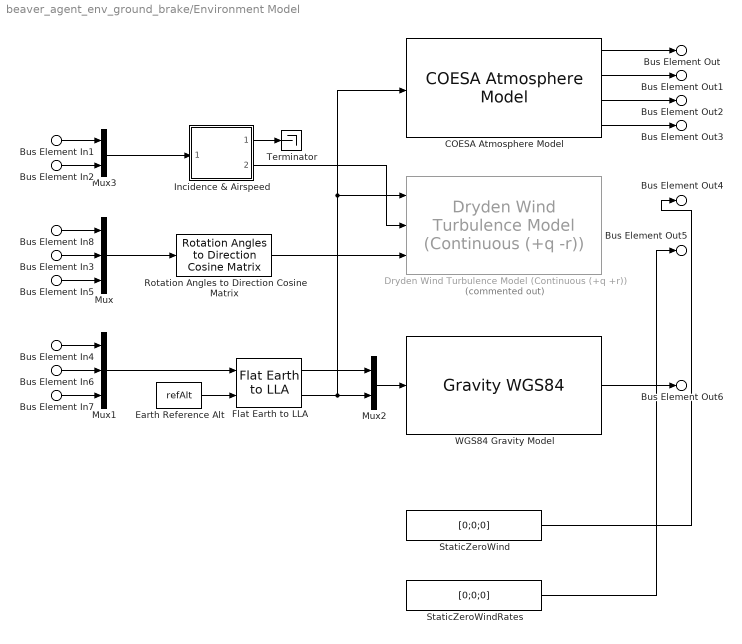
== system beaver_agent_env_ground_brake/Environment Model ==
  Bus Element In1 : Inport  PortName=States  Element=u
  Bus Element In2 : Inport  PortName=States  Element=w
  Bus Element In3 : Inport  PortName=States  Element=theta
  Bus Element In4 : Inport  PortName=States  Element=Xe
  Bus Element In7 : Inport  PortName=States  Element=Ze
  Bus Element In8 : Inport  PortName=States  Element=phi
  Bus Element In5 : Inport  PortName=States  Element=psi
  Bus Element In6 : Inport  PortName=States  Element=Ye
  COESA Atmosphere Model : aerolibatmos2/COESA Atmosphere Model  units=Metric (MKS)  spec=1976 COESA-extended U.S. Standard Atmosphere  model=Profile  profile_var=High temperature  profile_percent=1%  profile_alt=5 km (16404 ft)  envelope_var=High temperature  envelope_percent=1%  action=Warning
  Dryden Wind Turbulence Model (Continuous (+q +r)) : aerolibwind2/Dryden Wind Turbulence Model  (Continuous (+q -r))  Commented=on  units=Metric (MKS)  spec=MIL-F-8785C  model=Continuous Dryden (+q -r)  W20=W20  Wdeg=Wdeg  TurbProb=10^-2 - Light  L_high=L_high  Wingspan=Wingspan  ts=ts  Seed=Seed  T_on=off
  Earth Reference Alt : Constant  Value=refAlt
  Flat Earth to LLA : aerolibtransform2/Flat Earth to LLA  units=Metric (MKS)  ptype=Earth (WGS84)  F=1/298.257223563  R=6378137  refPosPort=off  LL0=[0 0]  psi=0
  Incidence & Airspeed : Subsystem
  Mux : Mux  Inputs=3
  Mux1 : Mux  Inputs=3
  Mux2 : Mux  Inputs=2
  Mux3 : Mux  Inputs=2
  Rotation Angles to Direction Cosine Matrix : sharedtransform/Rotation Angles to Direction Cosine Matrix  rotationOrder=ZYX  aMode=aMode
      settings: SourceProductBaseCode=AE,PW,DR,MT,VE
  StaticZeroWind : Constant  Value=[0;0;0]
  StaticZeroWindRates : Constant  Value=[0;0;0]
  Terminator : Terminator
  "WGS84 Gravity Model  " : GravityWGS84
  Bus Element Out : Outport  VectorParamsAs1DForOutWhenUnconnected=off  PortName=Env  Element=To
  Bus Element Out1 : Outport  VectorParamsAs1DForOutWhenUnconnected=off  PortName=Env  Element=a
  Bus Element Out2 : Outport  VectorParamsAs1DForOutWhenUnconnected=off  PortName=Env  Element=Po
  Bus Element Out3 : Outport  VectorParamsAs1DForOutWhenUnconnected=off  PortName=Env  Element=AirDensity
  Bus Element Out4 : Outport  VectorParamsAs1DForOutWhenUnconnected=off  PortName=Env  Element=WindVelocity
  Bus Element Out5 : Outport  VectorParamsAs1DForOutWhenUnconnected=off  PortName=Env  Element=WindAngularRates
  Bus Element Out6 : Outport  VectorParamsAs1DForOutWhenUnconnected=off  PortName=Env  Element=g
  wires:
  Mux2/1 -> "WGS84 Gravity Model  "/1
  Bus Element In4/1 -> Mux1/1
  Bus Element In7/1 -> Mux1/3
  Bus Element In6/1 -> Mux1/2
  Bus Element In5/1 -> Mux/3
  Bus Element In8/1 -> Mux/1
  Bus Element In2/1 -> Mux3/2
  Bus Element In1/1 -> Mux3/1
  "WGS84 Gravity Model  "/1 -> Bus Element Out6/1
  COESA Atmosphere Model/2 -> Bus Element Out1/1
  COESA Atmosphere Model/1 -> Bus Element Out/1
  COESA Atmosphere Model/4 -> Bus Element Out3/1
  COESA Atmosphere Model/3 -> Bus Element Out2/1
  Flat Earth to LLA/1 -> Mux2/1
  Earth Reference Alt/1 -> Flat Earth to LLA/2
  Flat Earth to LLA/2 -> Mux2/2, COESA Atmosphere Model/1, Dryden Wind Turbulence Model (Continuous (+q +r))/1
  Mux3/1 -> Incidence & Airspeed/1(Velocity)
  Mux/1 -> Rotation Angles to Direction Cosine Matrix/1
  Bus Element In3/1 -> Mux/2
  Rotation Angles to Direction Cosine Matrix/1 -> Dryden Wind Turbulence Model (Continuous (+q +r))/3
  Mux1/1 -> Flat Earth to LLA/1
  StaticZeroWind/1 -> Bus Element Out4/1
  StaticZeroWindRates/1 -> Bus Element Out5/1
  Incidence & Airspeed/1(Alpha) -> Terminator/1
  Incidence & Airspeed/2(TrueAirspeed) -> Dryden Wind Turbulence Model (Continuous (+q +r))/2

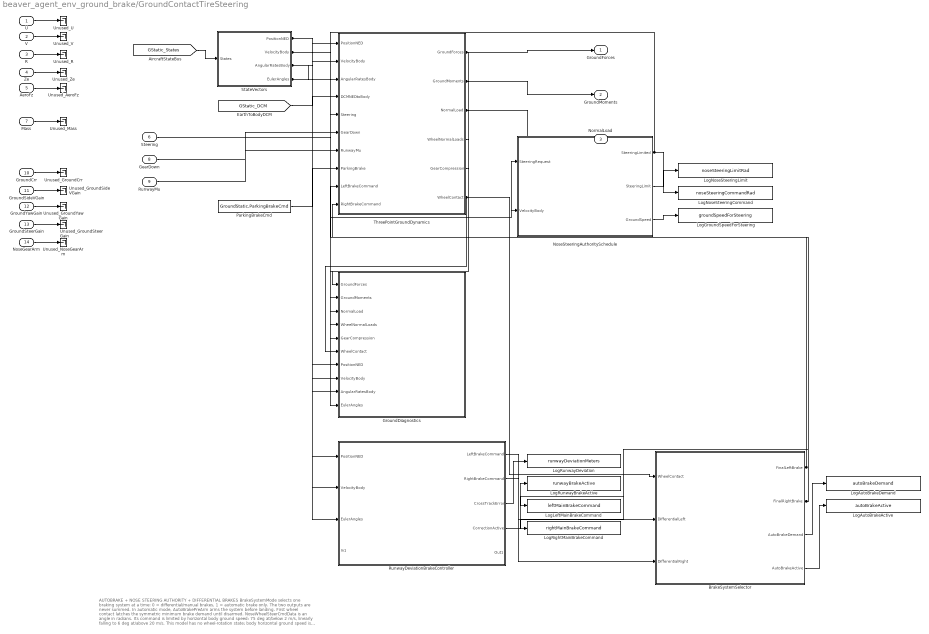
== system beaver_agent_env_ground_brake/GroundContactTireSteering ==
  note: AUTOBRAKE + NOSE STEERING AUTHORITY + DIFFERENTIAL BRAKES
      | BrakeSystemMode selects one braking system at a time: 0 = differential/manual brakes, 1 = automatic brake only. The two outputs are never summed.
      | In automatic mode, AutoBrakePreArm arms the system before landing. First wheel contact latches the symmetric minimum brake demand until disarmed.
      | NoseWheelSteerCmdData is an angle in radians. Its command is limited by horizontal body ground speed: 75 deg at/below 2 m/s, linearly falling to 6 deg at/above 20 m/s.
      | This model has no wheel-rotation state; body horizontal ground speed is the steering-schedule proxy. Parameters are demonstration values, not aircraft certification data.
  U : Inport
  V : Inport  Port=2
  R : Inport  Port=3
  Ze : Inport  Port=4
  AeroFz : Inport  Port=5
  Steering : Inport  Port=6
  Mass : Inport  Port=7
  GearDown : Inport  Port=8
  RunwayMu : Inport  Port=9
  GroundCrr : Inport  Port=10
  GroundSideVGain : Inport  Port=11
  GroundYawGain : Inport  Port=12
  GroundSteerGain : Inport  Port=13
  NoseGearArm : Inport  Port=14
  BrakeSystemSelector : Subsystem
  GroundDiagnostics : Subsystem
  LogAutoBrakeActive : ToWorkspace  VariableName=autoBrakeActive  SaveFormat=Timeseries  SampleTime=-1
  LogAutoBrakeDemand : ToWorkspace  VariableName=autoBrakeDemand  SaveFormat=Timeseries  SampleTime=-1
  LogGroundSpeedForSteering : ToWorkspace  VariableName=groundSpeedForSteering  SaveFormat=Timeseries  SampleTime=-1
  LogLeftMainBrakeCommand : ToWorkspace  VariableName=leftMainBrakeCommand  SaveFormat=Timeseries  SampleTime=-1
  LogNoseSteeringCommand : ToWorkspace  VariableName=noseSteeringCommandRad  SaveFormat=Timeseries  SampleTime=-1
  LogNoseSteeringLimit : ToWorkspace  VariableName=noseSteeringLimitRad  SaveFormat=Timeseries  SampleTime=-1
  LogRightMainBrakeCommand : ToWorkspace  VariableName=rightMainBrakeCommand  SaveFormat=Timeseries  SampleTime=-1
  LogRunwayBrakeActive : ToWorkspace  VariableName=runwayBrakeActive  SaveFormat=Timeseries  SampleTime=-1
  LogRunwayDeviation : ToWorkspace  VariableName=runwayDeviationMeters  SaveFormat=Timeseries  SampleTime=-1
  NoseSteeringAuthoritySchedule : Subsystem
  ParkingBrakeCmd : Constant  Value=GroundStatic.ParkingBrakeCmd
  RunwayDeviationBrakeController : Subsystem
  StateVectors : Subsystem
  ThreePointGroundDynamics : Subsystem
  Unused_AeroFz : Terminator
  Unused_GroundCrr : Terminator
  Unused_GroundSideVGain : Terminator
  Unused_GroundSteerGain : Terminator
  Unused_GroundYawGain : Terminator
  Unused_Mass : Terminator
  Unused_NoseGearArm : Terminator
  Unused_R : Terminator
  Unused_U : Terminator
  Unused_V : Terminator
  Unused_Ze : Terminator
  GroundForces : Outport
  GroundMoments : Outport  Port=2
  NormalLoad : Outport  Port=3
  wires:
  U/1 -> Unused_U/1
  V/1 -> Unused_V/1
  R/1 -> Unused_R/1
  Ze/1 -> Unused_Ze/1
  AeroFz/1 -> Unused_AeroFz/1
  Mass/1 -> Unused_Mass/1
  GroundCrr/1 -> Unused_GroundCrr/1
  GroundSideVGain/1 -> Unused_GroundSideVGain/1
  GroundYawGain/1 -> Unused_GroundYawGain/1
  GroundSteerGain/1 -> Unused_GroundSteerGain/1
  NoseGearArm/1 -> Unused_NoseGearArm/1
  [GStatic_States] -> StateVectors/1(States)
  StateVectors/1(PositionNED) -> ThreePointGroundDynamics/1(PositionNED), GroundDiagnostics/7(PositionNED), RunwayDeviationBrakeController/1(PositionNED)
  StateVectors/2(VelocityBody) -> ThreePointGroundDynamics/2(VelocityBody), GroundDiagnostics/8(VelocityBody), RunwayDeviationBrakeController/2(VelocityBody), NoseSteeringAuthoritySchedule/2(VelocityBody)
  StateVectors/3(AngularRatesBody) -> ThreePointGroundDynamics/3(AngularRatesBody), GroundDiagnostics/9(AngularRatesBody)
  [GStatic_DCM] -> ThreePointGroundDynamics/4(DCMNEDtoBody)
  Steering/1 -> NoseSteeringAuthoritySchedule/1(SteeringRequest)
  GearDown/1 -> ThreePointGroundDynamics/6(GearDown)
  RunwayMu/1 -> ThreePointGroundDynamics/7(RunwayMu)
  ParkingBrakeCmd/1 -> ThreePointGroundDynamics/8(ParkingBrake)
  ThreePointGroundDynamics/1(GroundForces) -> GroundForces/1, GroundDiagnostics/1(GroundForces)
  ThreePointGroundDynamics/2(GroundMoments) -> GroundMoments/1, GroundDiagnostics/2(GroundMoments)
  ThreePointGroundDynamics/3(NormalLoad) -> NormalLoad/1, GroundDiagnostics/3(NormalLoad)
  ThreePointGroundDynamics/4(WheelNormalLoads) -> GroundDiagnostics/4(WheelNormalLoads)
  ThreePointGroundDynamics/5(GearCompression) -> GroundDiagnostics/5(GearCompression)
  ThreePointGroundDynamics/6(WheelContact) -> GroundDiagnostics/6(WheelContact), BrakeSystemSelector/1(WheelContact)
  StateVectors/4(EulerAngles) -> GroundDiagnostics/10(EulerAngles), RunwayDeviationBrakeController/3(EulerAngles)
  RunwayDeviationBrakeController/1(LeftBrakeCommand) -> BrakeSystemSelector/2(DifferentialLeft)
  RunwayDeviationBrakeController/2(RightBrakeCommand) -> BrakeSystemSelector/3(DifferentialRight)
  RunwayDeviationBrakeController/3(CrossTrackError) -> LogRunwayDeviation/1
  RunwayDeviationBrakeController/4(CorrectionActive) -> LogRunwayBrakeActive/1
  NoseSteeringAuthoritySchedule/1(SteeringLimited) -> ThreePointGroundDynamics/5(Steering), LogNoseSteeringCommand/1
  BrakeSystemSelector/1(FinalLeftBrake) -> ThreePointGroundDynamics/9(LeftBrakeCommand), LogLeftMainBrakeCommand/1
  BrakeSystemSelector/2(FinalRightBrake) -> ThreePointGroundDynamics/10(RightBrakeCommand), LogRightMainBrakeCommand/1
  BrakeSystemSelector/3(AutoBrakeDemand) -> LogAutoBrakeDemand/1
  BrakeSystemSelector/4(AutoBrakeActive) -> LogAutoBrakeActive/1
  NoseSteeringAuthoritySchedule/2(SteeringLimit) -> LogNoseSteeringLimit/1
  NoseSteeringAuthoritySchedule/3(GroundSpeed) -> LogGroundSpeedForSteering/1

== system beaver_agent_env_ground_brake/Propulsion_Left ==
  cmd : Inport
  Gain : Gain  Gain=3.5
  Mux : Mux  Inputs=[1 2]
  Mux1 : Mux  Inputs=2
  ThrustX : Subsystem
  ThrustYZ : Constant  Value=[0 0]'  SampleTime=-1
  Thrust_M1 : Constant  Value=[0 0 0]'  SampleTime=-1
  Thrust_M2 : Constant  Value=[0 0]'  SampleTime=-1
  F : Outport  Unit=N  VectorParamsAs1DForOutWhenUnconnected=off
  M : Outport  Port=2  Unit=N*m  VectorParamsAs1DForOutWhenUnconnected=off
  wires:
  ThrustX/1(Thrust) -> Gain/1, Mux/1
  ThrustYZ/1 -> Mux/2
  Mux/1 -> F/1
  cmd/1 -> ThrustX/1(Throttle)
  Mux1/1 -> M/1
  Thrust_M2/1 -> Mux1/1
  Gain/1 -> Mux1/2

== system beaver_agent_env_ground_brake/Propulsion_Right ==
  cmd : Inport
  Gain : Gain  Gain=-3.5
  Mux : Mux  Inputs=[1 2]
  Mux1 : Mux  Inputs=2
  ThrustX : Subsystem
  ThrustYZ : Constant  Value=[0 0]'  SampleTime=-1
  Thrust_M1 : Constant  Value=[0 0 0]'  SampleTime=-1
  Thrust_M2 : Constant  Value=[0 0]'  SampleTime=-1
  F : Outport  Unit=N  VectorParamsAs1DForOutWhenUnconnected=off
  M : Outport  Port=2  Unit=N*m  VectorParamsAs1DForOutWhenUnconnected=off
  wires:
  ThrustX/1(Thrust) -> Gain/1, Mux/1
  ThrustYZ/1 -> Mux/2
  Mux/1 -> F/1
  cmd/1 -> ThrustX/1(Throttle)
  Mux1/1 -> M/1
  Thrust_M2/1 -> Mux1/1
  Gain/1 -> Mux1/2

== system beaver_agent_env_ground_brake/Visualization ==
  Bus Element In : Inport  PortName=States  Element=u
  Bus Element In1 : Inport  PortName=States  Element=w
  Bus Element In3 : Inport  PortName=States  Element=q
  Bus Element In4 : Inport  PortName=States  Element=theta
  Bus Element In12 : Inport  PortName=States  Element=Ze
  Bus Element In2 : Inport  PortName=States  Element=Xe
  Bus Element In10 : Inport  PortName=States  Element=v
  Bus Element In5 : Inport  PortName=States  Element=phi
  Bus Element In6 : Inport  PortName=States  Element=psi
  Bus Element In7 : Inport  PortName=States  Element=p
  Bus Element In8 : Inport  PortName=States  Element=r
  Bus Element In9 : Inport  PortName=States  Element=Ye
  "Incidence, Sideslip, & Airspeed" : Subsystem
  LogDisplayAttitude : ToWorkspace  VariableName=visualizationAttitude  SaveFormat=Timeseries  SampleTime=-1
  LogDisplayIncidence : ToWorkspace  VariableName=visualizationIncidence  SaveFormat=Timeseries  SampleTime=-1
  LogDisplayPosition : ToWorkspace  VariableName=visualizationPosition  SaveFormat=Timeseries  SampleTime=-1
  LogDisplayRates : ToWorkspace  VariableName=visualizationRates  SaveFormat=Timeseries  SampleTime=-1
  Mux{1..4} (4 alike) : Mux  Inputs=3
  Mux5 : Mux  Inputs=2
  State Plots : Scope  NumInputPorts=4
  Terminator : Terminator
  wires:
  Mux3/1 -> State Plots/4, LogDisplayPosition/1
  Bus Element In2/1 -> Mux3/1  "Xe"
  Bus Element In9/1 -> Mux3/2  "Ye"
  Bus Element In12/1 -> Mux3/3  "Ze"
  Mux2/1 -> State Plots/3, LogDisplayRates/1
  Mux1/1 -> State Plots/2, LogDisplayAttitude/1
  Mux5/1 -> State Plots/1, LogDisplayIncidence/1
  Bus Element In10/1 -> Mux4/2
  Bus Element In8/1 -> Mux2/3  "r"
  Bus Element In7/1 -> Mux2/1  "p"
  Bus Element In6/1 -> Mux1/3  "psi"
  Bus Element In5/1 -> Mux1/1  "phi"
  Bus Element In4/1 -> Mux1/2  "theta"
  Bus Element In3/1 -> Mux2/2  "q"
  Bus Element In1/1 -> Mux4/3
  Bus Element In/1 -> Mux4/1
  Mux4/1 -> "Incidence, Sideslip, & Airspeed"/1(Velocity)
  "Incidence, Sideslip, & Airspeed"/1(Alpha) -> Mux5/1  "alpha"
  "Incidence, Sideslip, & Airspeed"/2(Beta) -> Mux5/2  "beta"
  "Incidence, Sideslip, & Airspeed"/3(TrueAirspeed) -> Terminator/1

== system beaver_agent_env_ground_brake/Aerodynamic Model/Actuator Aerodynamic Coefficients ==
  Bus Element In13 : Inport  PortName=ActuatorCmds  Element=Elevator
  Bus Element In1 : Inport  PortName=ActuatorCmds  Element=Aileron
  Bus Element In2 : Inport  PortName=ActuatorCmds  Element=Rudder
  Alpha : Inport  Port=2
  Beta2 : Inport  Port=3
  Aileron : Subsystem
  Elevator : Subsystem
  Flap : Subsystem
  In Bus Element : Constant  Value=0
      settings: AttributesFormatString=Flap = 0
  Rudder : Subsystem
  Sum : Sum  Inputs=4  InputSameDT=on  SaturateOnIntegerOverflow=on  OutDataTypeStr=Inherit: Same as first input
  Coeff : Outport  InitialOutput=0  VectorParamsAs1DForOutWhenUnconnected=off
  wires:
  Bus Element In2/1 -> Rudder/1(Actuator)
  Bus Element In1/1 -> Aileron/1(Actuator)
  Bus Element In13/1 -> Elevator/1(Actuator)
  Beta2/1 -> Elevator/2(Beta2)
  Flap/1(delCoeff) -> Sum/4
  Alpha/1 -> Flap/2(Alpha), Rudder/2(Alpha), Aileron/2(Alpha)
  Rudder/1(delCoeff) -> Sum/3
  Aileron/1(delCoeff) -> Sum/2
  Elevator/1(delCoeff) -> Sum/1
  Sum/1 -> Coeff/1
  In Bus Element/1 -> Flap/1(Actuator)

== system beaver_agent_env_ground_brake/Aerodynamic Model/Aerodynamic Coefficients ==
  Alpha : Inport
  Alpha2 : Inport  Port=2
  Alpha3 : Inport  Port=3
  Beta : Inport  Port=4
  Beta2 : Inport  Port=5
  Beta3 : Inport  Port=6
  V : Inport  Port=7
  pqr : Inport  Port=8  Unit=m/s
  Body Rate Damping : Subsystem
  Datum Coefficients : Subsystem
  Sum : Sum  Inputs=|++
  Coeff : Outport  VectorParamsAs1DForOutWhenUnconnected=off
  wires:
  pqr/1 -> Body Rate Damping/2(pqr)
  Sum/1 -> Coeff/1
  V/1 -> Body Rate Damping/1(V)
  Body Rate Damping/1(Coeff) -> Sum/2
  Datum Coefficients/1(Coeff) -> Sum/1
  Beta/1 -> Datum Coefficients/4(Beta)
  Alpha/1 -> Datum Coefficients/1(Alpha)
  Alpha2/1 -> Datum Coefficients/2(Alpha2)
  Alpha3/1 -> Datum Coefficients/3(Alpha3)
  Beta2/1 -> Datum Coefficients/5(Beta2)
  Beta3/1 -> Datum Coefficients/6(Beta3)

== system beaver_agent_env_ground_brake/Aerodynamic Model/Subsystem ==
  Vb : Inport
  "Incidence, Sideslip, & Airspeed" : Subsystem
  Product{,1..3} (4 alike) : Product
  Alpha : Outport
  Alpha2 : Outport  Port=2
  Alpha3 : Outport  Port=3
  Beta : Outport  Port=4
  Beta2 : Outport  Port=5
  Beta3 : Outport  Port=6
  V : Outport  Port=7
  wires:
  Product/1 -> Product1/1, Alpha2/1
  Vb/1 -> "Incidence, Sideslip, & Airspeed"/1(Velocity)
  Product1/1 -> Alpha3/1
  Product2/1 -> Product3/1, Beta2/1
  Product3/1 -> Beta3/1
  "Incidence, Sideslip, & Airspeed"/1(Alpha) -> Product/1, Alpha/1, Product/2, Product1/2
  "Incidence, Sideslip, & Airspeed"/2(Beta) -> Product3/2, Product2/2, Product2/1, Beta/1
  "Incidence, Sideslip, & Airspeed"/3(TrueAirspeed) -> V/1

== system beaver_agent_env_ground_brake/Aerodynamic Model/ToBus ==
  I : Inport
  Bus Creator3 : BusCreator  Inputs=3
  Demux : Demux  Outputs=3
  O : Outport  VectorParamsAs1DForOutWhenUnconnected=off
  wires:
  I/1 -> Demux/1
  Demux/2 -> Bus Creator3/2  "q_wind"
  Bus Creator3/1 -> O/1
  Demux/3 -> Bus Creator3/3  "r_wind"
  Demux/1 -> Bus Creator3/1  "p_wind"

== system beaver_agent_env_ground_brake/Environment Model/Incidence & Airspeed ==
  Velocity : Inport
  AngleOfAttack : Trigonometry  Operator=atan2
  Components : Demux  Outputs=2
  Speed : Sqrt
  SpeedSquared : Sum
  V1Squared : Product  Inputs=**
  V2Squared : Product  Inputs=**
  Alpha : Outport
  TrueAirspeed : Outport  Port=2
  wires:
  Speed/1 -> TrueAirspeed/1
  AngleOfAttack/1 -> Alpha/1
  V1Squared/1 -> SpeedSquared/1
  SpeedSquared/1 -> Speed/1
  V2Squared/1 -> SpeedSquared/2
  Velocity/1 -> Components/1
  Components/2 -> V2Squared/1, V2Squared/2, AngleOfAttack/1
  Components/1 -> V1Squared/1, V1Squared/2, AngleOfAttack/2

== system beaver_agent_env_ground_brake/GroundContactTireSteering/BrakeSystemSelector ==
  WheelContact : Inport
  DifferentialLeft : Inport  Port=2
  DifferentialRight : Inport  Port=3
  AnyWheelContact : Logic  Operator=OR  Inputs=3  AllPortsSameDT=off  OutDataTypeStr=boolean
  AutoBrakeEnabled : Logic  Inputs=3  AllPortsSameDT=off  OutDataTypeStr=boolean
  AutoBrakeModeBoolean : simulink/Logic and Bit Operations/Compare To Constant  relop===  const=1  OutDataTypeStr=boolean
  BrakeSystemModeSetting : Constant  Value=GroundStatic.BrakeSystemMode
  LandingContactLatch : Memory
  LandingDetected : Logic  Operator=OR  AllPortsSameDT=off  OutDataTypeStr=boolean
  LeftFinalLimit : Saturate  UpperLimit=1  LowerLimit=0
  MinimumAutoBrakeDemand : Switch  Criteria=u2 ~= 0  SaturateOnIntegerOverflow=off  InputSameDT=off
  MinimumBrakeLimit : Saturate  UpperLimit=1  LowerLimit=0
  MinimumBrakeSetting : Constant  Value=GroundStatic.AutoBrakeMinLevel
  PreArmBoolean : simulink/Logic and Bit Operations/Compare To Constant  relop=~=  const=0  OutDataTypeStr=boolean
  PreArmSetting : Constant  Value=GroundStatic.AutoBrakePreArm
  RightFinalLimit : Saturate  UpperLimit=1  LowerLimit=0
  SelectLeftBrakeSystem : Switch  Criteria=u2 ~= 0  SaturateOnIntegerOverflow=off  InputSameDT=off
  SelectRightBrakeSystem : Switch  Criteria=u2 ~= 0  SaturateOnIntegerOverflow=off  InputSameDT=off
  Wheel1ContactBoolean : simulink/Logic and Bit Operations/Compare To Constant  relop=>  const=0.5  OutDataTypeStr=boolean
  Wheel2ContactBoolean : simulink/Logic and Bit Operations/Compare To Constant  relop=>  const=0.5  OutDataTypeStr=boolean
  Wheel3ContactBoolean : simulink/Logic and Bit Operations/Compare To Constant  relop=>  const=0.5  OutDataTypeStr=boolean
  WheelContacts : Demux  Outputs=3
  ZeroBrake : Constant  Value=0
  FinalLeftBrake : Outport
  FinalRightBrake : Outport  Port=2
  AutoBrakeDemand : Outport  Port=3
  AutoBrakeActive : Outport  Port=4
  wires:
  ? -> ?
  WheelContact/1 -> WheelContacts/1
  WheelContacts/1 -> Wheel1ContactBoolean/1
  WheelContacts/2 -> Wheel2ContactBoolean/1
  WheelContacts/3 -> Wheel3ContactBoolean/1
  Wheel1ContactBoolean/1 -> AnyWheelContact/1
  Wheel2ContactBoolean/1 -> AnyWheelContact/2
  Wheel3ContactBoolean/1 -> AnyWheelContact/3
  PreArmSetting/1 -> PreArmBoolean/1
  BrakeSystemModeSetting/1 -> AutoBrakeModeBoolean/1
  AnyWheelContact/1 -> LandingDetected/1
  LandingContactLatch/1 -> LandingDetected/2
  LandingDetected/1 -> AutoBrakeEnabled/1
  PreArmBoolean/1 -> AutoBrakeEnabled/2
  AutoBrakeModeBoolean/1 -> AutoBrakeEnabled/3, SelectLeftBrakeSystem/2, SelectRightBrakeSystem/2
  AutoBrakeEnabled/1 -> LandingContactLatch/1, MinimumAutoBrakeDemand/2, AutoBrakeActive/1
  MinimumBrakeSetting/1 -> MinimumBrakeLimit/1
  MinimumBrakeLimit/1 -> MinimumAutoBrakeDemand/1
  ZeroBrake/1 -> MinimumAutoBrakeDemand/3
  MinimumAutoBrakeDemand/1 -> AutoBrakeDemand/1, SelectLeftBrakeSystem/1, SelectRightBrakeSystem/1
  SelectLeftBrakeSystem/1 -> LeftFinalLimit/1
  SelectRightBrakeSystem/1 -> RightFinalLimit/1
  LeftFinalLimit/1 -> FinalLeftBrake/1
  RightFinalLimit/1 -> FinalRightBrake/1
  DifferentialLeft/1 -> SelectLeftBrakeSystem/3
  DifferentialRight/1 -> SelectRightBrakeSystem/3

== system beaver_agent_env_ground_brake/GroundContactTireSteering/GroundDiagnostics ==
  GroundForces : Inport
  GroundMoments : Inport  Port=2
  NormalLoad : Inport  Port=3
  WheelNormalLoads : Inport  Port=4
  GearCompression : Inport  Port=5
  WheelContact : Inport  Port=6
  PositionNED : Inport  Port=7
  VelocityBody : Inport  Port=8
  AngularRatesBody : Inport  Port=9
  EulerAngles : Inport  Port=10
  LogAngularRatesBody : ToWorkspace  VariableName=groundAngularRates  SaveFormat=Timeseries  SampleTime=-1
  LogEulerAngles : ToWorkspace  VariableName=groundEulerAngles  SaveFormat=Timeseries  SampleTime=-1
  LogGearCompression : ToWorkspace  VariableName=gearCompression  SaveFormat=Timeseries  SampleTime=-1
  LogGroundForces : ToWorkspace  VariableName=groundForcesDetailed  SaveFormat=Timeseries  SampleTime=-1
  LogGroundMoments : ToWorkspace  VariableName=groundMomentsDetailed  SaveFormat=Timeseries  SampleTime=-1
  LogNormalLoad : ToWorkspace  VariableName=groundNormalLoadDetailed  SaveFormat=Timeseries  SampleTime=-1
  LogPositionNED : ToWorkspace  VariableName=groundPositionNED  SaveFormat=Timeseries  SampleTime=-1
  LogVelocityBody : ToWorkspace  VariableName=groundVelocityBody  SaveFormat=Timeseries  SampleTime=-1
  LogWheelContact : ToWorkspace  VariableName=wheelContact  SaveFormat=Timeseries  SampleTime=-1
  LogWheelNormalLoads : ToWorkspace  VariableName=wheelNormalLoads  SaveFormat=Timeseries  SampleTime=-1
  wires:
  GroundForces/1 -> LogGroundForces/1
  GroundMoments/1 -> LogGroundMoments/1
  NormalLoad/1 -> LogNormalLoad/1
  WheelNormalLoads/1 -> LogWheelNormalLoads/1
  GearCompression/1 -> LogGearCompression/1
  WheelContact/1 -> LogWheelContact/1
  PositionNED/1 -> LogPositionNED/1
  VelocityBody/1 -> LogVelocityBody/1
  AngularRatesBody/1 -> LogAngularRatesBody/1
  EulerAngles/1 -> LogEulerAngles/1

== system beaver_agent_env_ground_brake/GroundContactTireSteering/NoseSteeringAuthoritySchedule ==
  SteeringRequest : Inport
  VelocityBody : Inport  Port=2
  AngleRange : Gain  Gain=GroundStatic.NoseSteerAngleHighSpeed-GroundStatic.NoseSteerAngleLowSpeed
  ForwardSpeedSquared : Product  Inputs=**
  GroundSpeedMagnitude : Sqrt
  HighScheduleSpeed : Constant  Value=GroundStatic.NoseSteerHighSpeed
  HorizontalSpeedSquared : Sum
  LateralSpeedSquared : Product  Inputs=**
  LimitScheduleFraction : Saturate  UpperLimit=1  LowerLimit=0
  LowScheduleSpeed : Constant  Value=GroundStatic.NoseSteerLowSpeed
  LowSpeedMaxAngle : Constant  Value=GroundStatic.NoseSteerAngleLowSpeed
  LowerSteeringClamp : MinMax  Function=max  Inputs=2
  NegativeAngleLimit : Gain  Gain=-1
  NormalizeSpeedRange : Gain  Gain=1/(GroundStatic.NoseSteerHighSpeed-GroundStatic.NoseSteerLowSpeed)
  ScheduledAngleLimit : Sum
  SpeedAboveLowThreshold : Sum  Inputs=+-
  UpperSteeringClamp : MinMax  Inputs=2
  VelocityComponents : Demux  Outputs=3
  SteeringLimited : Outport
  SteeringLimit : Outport  Port=2
  GroundSpeed : Outport  Port=3
  wires:
  ? -> ?
  VelocityBody/1 -> VelocityComponents/1
  VelocityComponents/1 -> ForwardSpeedSquared/1, ForwardSpeedSquared/2
  VelocityComponents/2 -> LateralSpeedSquared/1, LateralSpeedSquared/2
  ForwardSpeedSquared/1 -> HorizontalSpeedSquared/1
  LateralSpeedSquared/1 -> HorizontalSpeedSquared/2
  HorizontalSpeedSquared/1 -> GroundSpeedMagnitude/1
  GroundSpeedMagnitude/1 -> SpeedAboveLowThreshold/1, GroundSpeed/1
  LowScheduleSpeed/1 -> SpeedAboveLowThreshold/2
  SpeedAboveLowThreshold/1 -> NormalizeSpeedRange/1
  NormalizeSpeedRange/1 -> LimitScheduleFraction/1
  LimitScheduleFraction/1 -> AngleRange/1
  LowSpeedMaxAngle/1 -> ScheduledAngleLimit/1
  AngleRange/1 -> ScheduledAngleLimit/2
  SteeringRequest/1 -> UpperSteeringClamp/1
  ScheduledAngleLimit/1 -> UpperSteeringClamp/2, NegativeAngleLimit/1, SteeringLimit/1
  UpperSteeringClamp/1 -> LowerSteeringClamp/1
  NegativeAngleLimit/1 -> LowerSteeringClamp/2
  LowerSteeringClamp/1 -> SteeringLimited/1

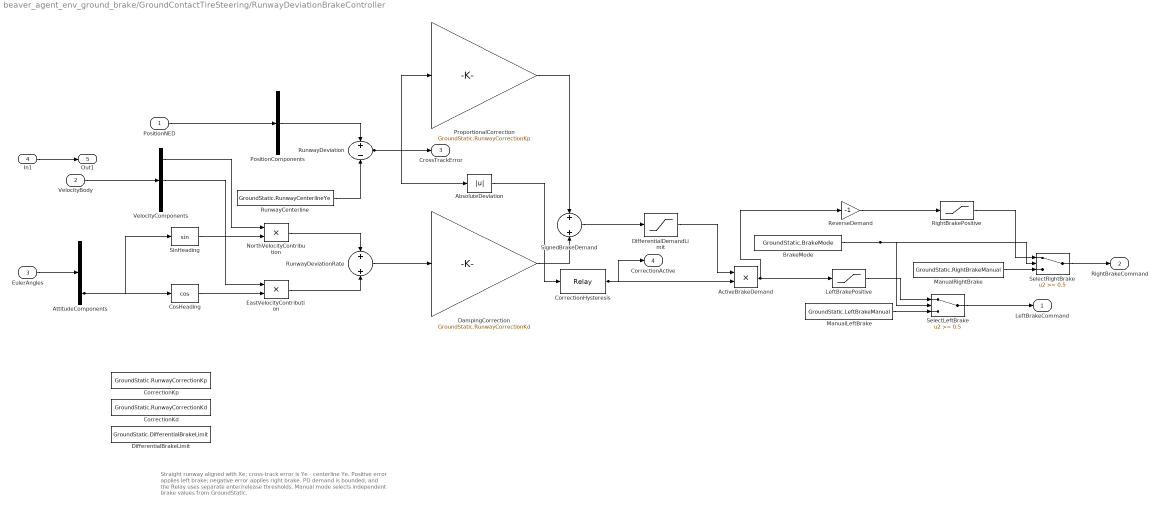
== system beaver_agent_env_ground_brake/GroundContactTireSteering/RunwayDeviationBrakeController ==
  note: Straight runway aligned with Xe; cross-track error is Ye - centerline Ye.
      | Positive error applies left brake; negative error applies right brake.
      | PD demand is bounded, and the Relay uses separate enter/release thresholds.
      | Manual mode selects independent brake values from GroundStatic.
  PositionNED : Inport
  VelocityBody : Inport  Port=2
  EulerAngles : Inport  Port=3
  In1 : Inport  Port=4
  AbsoluteDeviation : Abs  SaturateOnIntegerOverflow=off
  ActiveBrakeDemand : Product  Inputs=**
  AttitudeComponents : Demux  Outputs=3
  BrakeMode : Constant  Value=GroundStatic.BrakeMode
  CorrectionHysteresis : Relay  OnSwitchValue=GroundStatic.RunwayCorrectionOnThreshold  OffSwitchValue=GroundStatic.RunwayCorrectionOffThreshold
  CorrectionKd : Constant  Value=GroundStatic.RunwayCorrectionKd
  CorrectionKp : Constant  Value=GroundStatic.RunwayCorrectionKp
  CosHeading : Trigonometry  Operator=cos
  DampingCorrection : Gain  Gain=GroundStatic.RunwayCorrectionKd
  DifferentialBrakeLimit : Constant  Value=GroundStatic.DifferentialBrakeLimit
  DifferentialDemandLimit : Saturate  UpperLimit=GroundStatic.DifferentialBrakeLimit  LowerLimit=-GroundStatic.DifferentialBrakeLimit
  EastVelocityContribution : Product  Inputs=**
  LeftBrakePositive : Saturate  UpperLimit=1  LowerLimit=0
  ManualLeftBrake : Constant  Value=GroundStatic.LeftBrakeManual
  ManualRightBrake : Constant  Value=GroundStatic.RightBrakeManual
  NorthVelocityContribution : Product  Inputs=**
  PositionComponents : Demux  Outputs=3
  ProportionalCorrection : Gain  Gain=GroundStatic.RunwayCorrectionKp
  ReverseDemand : Gain  Gain=-1
  RightBrakePositive : Saturate  UpperLimit=1  LowerLimit=0
  RunwayCenterline : Constant  Value=GroundStatic.RunwayCenterlineYe
  RunwayDeviation : Sum  Inputs=+-
  RunwayDeviationRate : Sum
  SelectLeftBrake : Switch  Threshold=0.5  SaturateOnIntegerOverflow=off  InputSameDT=off
  SelectRightBrake : Switch  Threshold=0.5  SaturateOnIntegerOverflow=off  InputSameDT=off
  SignedBrakeDemand : Sum
  SinHeading : Trigonometry
  VelocityComponents : Demux  Outputs=3
  LeftBrakeCommand : Outport
  RightBrakeCommand : Outport  Port=2
  CrossTrackError : Outport  Port=3
  CorrectionActive : Outport  Port=4
  Out1 : Outport  Port=5
  wires:
  DifferentialDemandLimit/1 -> ActiveBrakeDemand/1
  RightBrakePositive/1 -> SelectRightBrake/1
  SelectRightBrake/1 -> RightBrakeCommand/1
  SelectLeftBrake/1 -> LeftBrakeCommand/1
  ManualRightBrake/1 -> SelectRightBrake/3
  ReverseDemand/1 -> RightBrakePositive/1
  ManualLeftBrake/1 -> SelectLeftBrake/3
  LeftBrakePositive/1 -> SelectLeftBrake/1
  SignedBrakeDemand/1 -> DifferentialDemandLimit/1
  DampingCorrection/1 -> SignedBrakeDemand/2
  ProportionalCorrection/1 -> SignedBrakeDemand/1
  RunwayDeviationRate/1 -> DampingCorrection/1
  AbsoluteDeviation/1 -> CorrectionHysteresis/1
  EastVelocityContribution/1 -> RunwayDeviationRate/2
  NorthVelocityContribution/1 -> RunwayDeviationRate/1
  CosHeading/1 -> EastVelocityContribution/2
  VelocityComponents/2 -> EastVelocityContribution/1
  SinHeading/1 -> NorthVelocityContribution/2
  VelocityComponents/1 -> NorthVelocityContribution/1
  RunwayCenterline/1 -> RunwayDeviation/2
  PositionComponents/2 -> RunwayDeviation/1
  EulerAngles/1 -> AttitudeComponents/1
  VelocityBody/1 -> VelocityComponents/1
  PositionNED/1 -> PositionComponents/1
  In1/1 -> Out1/1
  BrakeMode/1 -> SelectLeftBrake/2, SelectRightBrake/2
  ActiveBrakeDemand/1 -> LeftBrakePositive/1, ReverseDemand/1
  CorrectionHysteresis/1 -> ActiveBrakeDemand/2, CorrectionActive/1
  RunwayDeviation/1 -> AbsoluteDeviation/1, ProportionalCorrection/1, CrossTrackError/1
  AttitudeComponents/3 -> SinHeading/1, CosHeading/1

== system beaver_agent_env_ground_brake/GroundContactTireSteering/StateVectors ==
  States : Inport
  SelectStates : BusSelector  OutputSignals=Xe,Ye,Ze,u,v,w,p,q,r,phi,theta,psi
  Vector{1..4} (4 alike) : Mux  Inputs=3
  PositionNED : Outport
  VelocityBody : Outport  Port=2
  AngularRatesBody : Outport  Port=3
  EulerAngles : Outport  Port=4
  wires:
  Vector4/1 -> EulerAngles/1
  SelectStates/7 -> Vector3/1  "<p>"
  SelectStates/8 -> Vector3/2  "<q>"
  Vector1/1 -> PositionNED/1
  SelectStates/9 -> Vector3/3  "<r>"
  SelectStates/11 -> Vector4/2  "<theta>"
  Vector3/1 -> AngularRatesBody/1
  Vector2/1 -> VelocityBody/1
  SelectStates/10 -> Vector4/1  "<phi>"
  SelectStates/4 -> Vector2/1  "<u>"
  SelectStates/12 -> Vector4/3  "<psi>"
  SelectStates/6 -> Vector2/3  "<w>"
  SelectStates/5 -> Vector2/2  "<v>"
  SelectStates/3 -> Vector1/3  "<Ze>"
  States/1 -> SelectStates/1
  SelectStates/2 -> Vector1/2  "<Ye>"
  SelectStates/1 -> Vector1/1  "<Xe>"
